simulink model "beaver_agent_env_ground_static_preserved"  (R2022a)
settings: Solver=ode15s  StartTime=0.0  StopTime=30  FixedStep=1/120  MaxStep=0.005  RelTol=1e-6  AbsTol=1e-8
PreLoadFcn:
  | [aircraft, state] = astDehavillandBeaver();
  | thrustX = getCoefficient(aircraft,"CX","Propeller",Component="Propeller");
  | AileronCmd = 0.00202547955338193;
  | ElevatorCmd = -0.0109658218633661;
  | RudderCmd = -0.0374364069557001;
  | Throttle_Left = 0.16863024396043;
  | Throttle_Right = 0.16863024396043;
  | NoseWheelSteerCmdData = timeseries(0,0);
  | GearDownCmd = 1; RunwayMu = 0.65;
  | GroundMass = state.Mass;
  | GroundCrr = 0.015; GroundSideVGain = 0.35;
  | GroundYawGain = 0.15; GroundSteerGain = 0.8; NoseGearArm = 2.4;
  | 
  | Throttle_Left=0; Throttle_Right=0;
  | AileronCmd=0; ElevatorCmd=0; RudderCmd=0;
  | NoseWheelSteerCmdData=timeseries([0;0],[0;60]);
model workspace (MATLAB code in the model file + MAT data in the model file):
  GroundStatic : object (value not decoded)
  inputs0 : object (value not decoded)
  states : object (value not decoded)
  states0 : object (value not decoded)
  other statements: initialize6DOFSkyHogg;
values from neighbouring files (symbols this model uses):
  r = vec(out.r)    [ground_realtime_worker.m]    (also in probe_brake_correction.m; verify_ground_brake_model.m = runCase('turn_right_10',g,10,8))
  state = squeeze(controls.Data)    [finalize_ground_capability_checks.m]    (also in run_ground_capability_checks.m)
symbols that are objects in the model workspace (value not decoded): GroundStatic
undefined symbols (not defined in the file or in its folder): aircraft, Earth, F, Light, MIL, WGS84
libraries: shared6dof x1, aerolibadyn x1, aerolibasang x1, aerolibatmos2 x1, aerolibwind2 x1, aerolibtransform2 x1, sharedtransform x1
(part 2 of 2)

== system beaver_agent_env_ground_static_preserved/GroundContactTireSteering/ThreePointGroundDynamics/LeftMainGear ==
  PositionNED : Inport
  VelocityBody : Inport  Port=2
  AngularRatesBody : Inport  Port=3
  DCMNEDtoBody : Inport  Port=4
  Steering : Inport  Port=5
  GearDown : Inport  Port=6
  RunwayMu : Inport  Port=7
  ParkingBrake : Inport  Port=8
  ContactGeometry : Subsystem
  ContactMoment : Subsystem
  ForceResolution : Subsystem
  NormalReaction : Subsystem
  TireFrictionCircle : Subsystem
  WheelKinematics : Subsystem
  ForceBody : Outport
  MomentBody : Outport  Port=2
  NormalLoad : Outport  Port=3
  Compression : Outport  Port=4
  Contact : Outport  Port=5
  wires:
  ContactMoment/1(AxB) -> MomentBody/1
  ForceResolution/1(BodyForce_1) -> ContactMoment/2(B), ForceBody/1
  PositionNED/1 -> ContactGeometry/1(PositionNED)
  NormalReaction/1(NormalForce_1) -> NormalLoad/1, TireFrictionCircle/6(NormalForce_1), ForceResolution/8(NormalForce), TireFrictionCircle/4(NormalForce)
  AngularRatesBody/1 -> ContactGeometry/5(AngularRatesBody)
  ContactGeometry/5(PositiveCompression_1) -> Compression/1, NormalReaction/3(PositiveCompression)
  NormalReaction/2(ActiveContact_1) -> Contact/1
  ContactGeometry/6(ContactVelocityNED_1) -> WheelKinematics/6(ContactVelocityNED)
  GearDown/1 -> NormalReaction/4(GearDown)
  ContactGeometry/8(ContactGate_1) -> NormalReaction/2(ContactGate)
  ContactGeometry/7(CompressionRate_1) -> NormalReaction/1(CompressionRate)
  ContactGeometry/1(LoadedContactArm_1) -> ContactMoment/1(A)
  Steering/1 -> WheelKinematics/2(Steering)
  ParkingBrake/1 -> TireFrictionCircle/1(ParkingBrake)
  ContactGeometry/2(BodyToNED_1) -> WheelKinematics/3(BodyToNED)
  WheelKinematics/3(WheelLongVelocity_1) -> TireFrictionCircle/2(WheelLongVelocity)
  TireFrictionCircle/2(SideTireForce_1) -> ForceResolution/6(SideTireForce)
  ContactGeometry/3(Zero_1) -> WheelKinematics/4(Zero)
  VelocityBody/1 -> ContactGeometry/4(VelocityBody)
  WheelKinematics/4(WheelSideVelocity_1) -> TireFrictionCircle/3(WheelSideVelocity)
  RunwayMu/1 -> TireFrictionCircle/5(RunwayMu)
  TireFrictionCircle/1(LongTireForce_1) -> ForceResolution/5(LongTireForce)
  WheelKinematics/1(ForwardY_3) -> WheelKinematics/7(ForwardY_2), ForceResolution/7(ForwardY_1), WheelKinematics/1(ForwardY_1), ForceResolution/1(ForwardY)
  WheelKinematics/2(ForwardX_2) -> WheelKinematics/5(ForwardX_1), ForceResolution/2(ForwardX), ForceResolution/4(ForwardX_1)
  DCMNEDtoBody/1 -> ContactGeometry/2(DCMNEDtoBody), ForceResolution/3(DCMNEDtoBody), ContactGeometry/3(DCMNEDtoBody_1)

== system beaver_agent_env_ground_static_preserved/GroundContactTireSteering/ThreePointGroundDynamics/NoseGear ==
  PositionNED : Inport
  VelocityBody : Inport  Port=2
  AngularRatesBody : Inport  Port=3
  DCMNEDtoBody : Inport  Port=4
  Steering : Inport  Port=5
  GearDown : Inport  Port=6
  RunwayMu : Inport  Port=7
  ParkingBrake : Inport  Port=8
  ContactGeometry : Subsystem
  ContactMoment : Subsystem
  ForceResolution : Subsystem
  NormalReaction : Subsystem
  TireFrictionCircle : Subsystem
  WheelKinematics : Subsystem
  ForceBody : Outport
  MomentBody : Outport  Port=2
  NormalLoad : Outport  Port=3
  Compression : Outport  Port=4
  Contact : Outport  Port=5
  wires:
  DCMNEDtoBody/1 -> ContactGeometry/5(DCMNEDtoBody_1), ForceResolution/7(DCMNEDtoBody), ContactGeometry/4(DCMNEDtoBody)
  AngularRatesBody/1 -> ContactGeometry/3(AngularRatesBody)
  ContactMoment/1(AxB) -> MomentBody/1
  ContactGeometry/5(CompressionRate_1) -> NormalReaction/2(CompressionRate)
  PositionNED/1 -> ContactGeometry/1(PositionNED)
  VelocityBody/1 -> ContactGeometry/2(VelocityBody)
  NormalReaction/2(ActiveContact_1) -> Contact/1
  ContactGeometry/6(LoadedContactArm_1) -> ContactMoment/1(A)
  GearDown/1 -> NormalReaction/1(GearDown)
  Steering/1 -> WheelKinematics/2(Steering)
  ContactGeometry/2(ContactVelocityNED_1) -> WheelKinematics/3(ContactVelocityNED)
  ContactGeometry/3(BodyToNED_1) -> WheelKinematics/4(BodyToNED)
  WheelKinematics/1(ForwardY_2) -> ForceResolution/1(ForwardY), WheelKinematics/1(ForwardY_1), ForceResolution/2(ForwardY_1)
  ParkingBrake/1 -> TireFrictionCircle/5(ParkingBrake)
  RunwayMu/1 -> TireFrictionCircle/1(RunwayMu)
  WheelKinematics/3(WheelLongVelocity_1) -> TireFrictionCircle/2(WheelLongVelocity)
  WheelKinematics/4(WheelSideVelocity_1) -> TireFrictionCircle/3(WheelSideVelocity)
  WheelKinematics/2(ForwardX_1) -> ForceResolution/3(ForwardX)
  ContactGeometry/7(ContactGate_1) -> NormalReaction/3(ContactGate)
  ForceResolution/1(BodyForce_1) -> ContactMoment/2(B), ForceBody/1
  ContactGeometry/4(Zero_1) -> WheelKinematics/5(Zero)
  TireFrictionCircle/1(SideTireForce_1) -> ForceResolution/4(SideTireForce)
  TireFrictionCircle/2(LongTireForce_1) -> ForceResolution/5(LongTireForce)
  ContactGeometry/8(PositiveCompression_1) -> NormalReaction/4(PositiveCompression), Compression/1
  NormalReaction/1(NormalForce_1) -> NormalLoad/1, TireFrictionCircle/4(NormalForce), TireFrictionCircle/6(NormalForce_1), ForceResolution/6(NormalForce)

== system beaver_agent_env_ground_static_preserved/GroundContactTireSteering/ThreePointGroundDynamics/RightMainGear ==
  PositionNED : Inport
  VelocityBody : Inport  Port=2
  AngularRatesBody : Inport  Port=3
  DCMNEDtoBody : Inport  Port=4
  Steering : Inport  Port=5
  GearDown : Inport  Port=6
  RunwayMu : Inport  Port=7
  ParkingBrake : Inport  Port=8
  ContactGeometry : Subsystem
  ContactMoment : Subsystem
  ForceResolution : Subsystem
  NormalReaction : Subsystem
  TireFrictionCircle : Subsystem
  WheelKinematics : Subsystem
  ForceBody : Outport
  MomentBody : Outport  Port=2
  NormalLoad : Outport  Port=3
  Compression : Outport  Port=4
  Contact : Outport  Port=5
  wires:
  Steering/1 -> WheelKinematics/2(Steering)
  PositionNED/1 -> ContactGeometry/1(PositionNED)
  GearDown/1 -> NormalReaction/4(GearDown)
  WheelKinematics/1(ForwardY_3) -> WheelKinematics/7(ForwardY_2), ForceResolution/7(ForwardY_1), WheelKinematics/1(ForwardY_1), ForceResolution/1(ForwardY)
  VelocityBody/1 -> ContactGeometry/4(VelocityBody)
  AngularRatesBody/1 -> ContactGeometry/5(AngularRatesBody)
  ContactGeometry/1(LoadedContactArm_1) -> ContactMoment/1(A)
  ContactGeometry/7(CompressionRate_1) -> NormalReaction/1(CompressionRate)
  ContactGeometry/8(ContactGate_1) -> NormalReaction/2(ContactGate)
  NormalReaction/2(ActiveContact_1) -> Contact/1
  TireFrictionCircle/1(LongTireForce_1) -> ForceResolution/5(LongTireForce)
  ContactGeometry/2(BodyToNED_1) -> WheelKinematics/3(BodyToNED)
  ContactGeometry/3(Zero_1) -> WheelKinematics/4(Zero)
  ParkingBrake/1 -> TireFrictionCircle/1(ParkingBrake)
  ContactMoment/1(AxB) -> MomentBody/1
  WheelKinematics/3(WheelLongVelocity_1) -> TireFrictionCircle/2(WheelLongVelocity)
  WheelKinematics/4(WheelSideVelocity_1) -> TireFrictionCircle/3(WheelSideVelocity)
  ContactGeometry/6(ContactVelocityNED_1) -> WheelKinematics/6(ContactVelocityNED)
  TireFrictionCircle/2(SideTireForce_1) -> ForceResolution/6(SideTireForce)
  RunwayMu/1 -> TireFrictionCircle/5(RunwayMu)
  DCMNEDtoBody/1 -> ContactGeometry/2(DCMNEDtoBody), ForceResolution/3(DCMNEDtoBody), ContactGeometry/3(DCMNEDtoBody_1)
  ContactGeometry/5(PositiveCompression_1) -> Compression/1, NormalReaction/3(PositiveCompression)
  WheelKinematics/2(ForwardX_2) -> WheelKinematics/5(ForwardX_1), ForceResolution/2(ForwardX), ForceResolution/4(ForwardX_1)
  ForceResolution/1(BodyForce_1) -> ContactMoment/2(B), ForceBody/1
  NormalReaction/1(NormalForce_1) -> NormalLoad/1, TireFrictionCircle/6(NormalForce_1), ForceResolution/8(NormalForce), TireFrictionCircle/4(NormalForce)

== system beaver_agent_env_ground_static_preserved/Aerodynamic Model/Aerodynamic Coefficients/Body Rate Damping/Subsystem ==
  V : Inport
  Constant1 : Constant  Value=aircraft.ReferenceSpan
  Constant2 : Constant  Value=aircraft.ReferenceLength
  Divide : Subsystem
  Gain1 : Gain  Gain=1/2
  Product : Subsystem
  cV : Outport
  b2V : Outport  Port=2
  wires:
  Product/1(NormalizedRate) -> cV/1
  Constant1/1 -> Gain1/1
  V/1 -> Divide/2(TrueAirspeed), Product/2(TrueAirspeed)
  Divide/1(NormalizedRate) -> b2V/1
  Constant2/1 -> Product/1(Numerator)
  Gain1/1 -> Divide/1(Numerator)

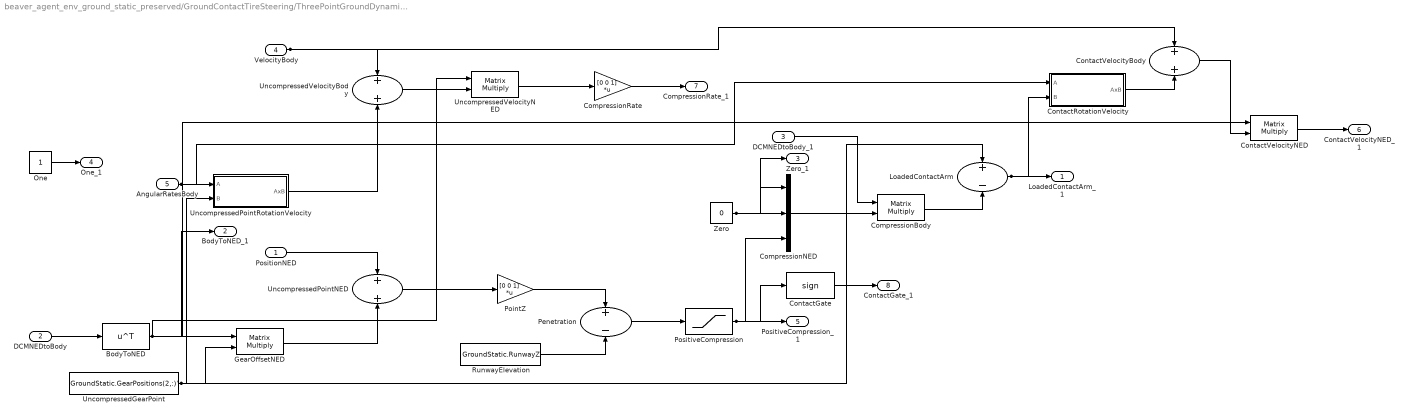
== system beaver_agent_env_ground_static_preserved/GroundContactTireSteering/ThreePointGroundDynamics/LeftMainGear/ContactGeometry ==
  PositionNED : Inport
  DCMNEDtoBody : Inport  Port=2
  DCMNEDtoBody_1 : Inport  Port=3
  VelocityBody : Inport  Port=4
  AngularRatesBody : Inport  Port=5
  BodyToNED : Math  Operator=transpose
  CompressionBody : Product  Inputs=**  Multiplication=Matrix(*)
  CompressionNED : Mux  Inputs=3
  CompressionRate : Gain  Gain=[0 0 1]  Multiplication=Matrix(K*u)
  ContactGate : Signum
  ContactRotationVelocity : Subsystem
  ContactVelocityBody : Sum
  ContactVelocityNED : Product  Inputs=**  Multiplication=Matrix(*)
  GearOffsetNED : Product  Inputs=**  Multiplication=Matrix(*)
  LoadedContactArm : Sum  Inputs=+-
  One : Constant
  Penetration : Sum  Inputs=+-
  PointZ : Gain  Gain=[0 0 1]  Multiplication=Matrix(K*u)
  PositiveCompression : Saturate  UpperLimit=inf  LowerLimit=0
  RunwayElevation : Constant  Value=GroundStatic.RunwayZ
  UncompressedGearPoint : Constant  Value=GroundStatic.GearPositions(2,:)'
  UncompressedPointNED : Sum
  UncompressedPointRotationVelocity : Subsystem
  UncompressedVelocityBody : Sum
  UncompressedVelocityNED : Product  Inputs=**  Multiplication=Matrix(*)
  Zero : Constant  Value=0
  LoadedContactArm_1 : Outport
  BodyToNED_1 : Outport  Port=2
  Zero_1 : Outport  Port=3
  One_1 : Outport  Port=4
  PositiveCompression_1 : Outport  Port=5
  ContactVelocityNED_1 : Outport  Port=6
  CompressionRate_1 : Outport  Port=7
  ContactGate_1 : Outport  Port=8
  wires:
  PositionNED/1 -> UncompressedPointNED/1
  ContactGate/1 -> ContactGate_1/1
  LoadedContactArm/1 -> ContactRotationVelocity/2(B), LoadedContactArm_1/1
  One/1 -> One_1/1
  CompressionRate/1 -> CompressionRate_1/1
  DCMNEDtoBody/1 -> BodyToNED/1
  Penetration/1 -> PositiveCompression/1
  ContactVelocityBody/1 -> ContactVelocityNED/2
  GearOffsetNED/1 -> UncompressedPointNED/2
  DCMNEDtoBody_1/1 -> CompressionBody/1
  UncompressedVelocityNED/1 -> CompressionRate/1
  PositiveCompression/1 -> PositiveCompression_1/1, ContactGate/1, CompressionNED/3
  UncompressedVelocityBody/1 -> UncompressedVelocityNED/2
  ContactRotationVelocity/1(AxB) -> ContactVelocityBody/2
  UncompressedPointRotationVelocity/1(AxB) -> UncompressedVelocityBody/2
  ContactVelocityNED/1 -> ContactVelocityNED_1/1
  UncompressedPointNED/1 -> PointZ/1
  CompressionBody/1 -> LoadedContactArm/2
  CompressionNED/1 -> CompressionBody/2
  PointZ/1 -> Penetration/1
  RunwayElevation/1 -> Penetration/2
  UncompressedGearPoint/1 -> LoadedContactArm/1, GearOffsetNED/2, UncompressedPointRotationVelocity/2(B)
  VelocityBody/1 -> ContactVelocityBody/1, UncompressedVelocityBody/1
  BodyToNED/1 -> ContactVelocityNED/1, GearOffsetNED/1, UncompressedVelocityNED/1, BodyToNED_1/1
  AngularRatesBody/1 -> ContactRotationVelocity/1(A), UncompressedPointRotationVelocity/1(A)
  Zero/1 -> CompressionNED/1, Zero_1/1, CompressionNED/2

== system beaver_agent_env_ground_static_preserved/GroundContactTireSteering/ThreePointGroundDynamics/LeftMainGear/ContactMoment ==
  A : Inport
  B : Inport  Port=2
  C1 : Sum  Inputs=+-
  C2 : Sum  Inputs=+-
  C3 : Sum  Inputs=+-
  DemuxA : Demux  Outputs=3
  DemuxB : Demux  Outputs=3
  N1 : Product  Inputs=**
  N2 : Product  Inputs=**
  N3 : Product  Inputs=**
  P1 : Product  Inputs=**
  P2 : Product  Inputs=**
  P3 : Product  Inputs=**
  Result : Mux  Inputs=3
  AxB : Outport
  wires:
  C1/1 -> Result/1
  Result/1 -> AxB/1
  P3/1 -> C3/1
  B/1 -> DemuxB/1
  C3/1 -> Result/3
  C2/1 -> Result/2
  N3/1 -> C3/2
  N2/1 -> C2/2
  P2/1 -> C2/1
  N1/1 -> C1/2
  P1/1 -> C1/1
  A/1 -> DemuxA/1
  DemuxA/2 -> P1/1, N3/1
  DemuxA/1 -> N2/1, P3/1
  DemuxB/2 -> N1/2, P3/2
  DemuxB/1 -> P2/2, N3/2
  DemuxA/3 -> N1/1, P2/1
  DemuxB/3 -> P1/2, N2/2

== system beaver_agent_env_ground_static_preserved/GroundContactTireSteering/ThreePointGroundDynamics/LeftMainGear/ForceResolution ==
  ForwardY : Inport
  ForwardX : Inport  Port=2
  DCMNEDtoBody : Inport  Port=3
  ForwardX_1 : Inport  Port=4
  LongTireForce : Inport  Port=5
  SideTireForce : Inport  Port=6
  ForwardY_1 : Inport  Port=7
  NormalForce : Inport  Port=8
  BodyForce : Product  Inputs=**  Multiplication=Matrix(*)
  FXLong : Product  Inputs=**
  FXSide : Product  Inputs=**
  FYLong : Product  Inputs=**
  FYSide : Product  Inputs=**
  ForceNED : Mux  Inputs=3
  ForceX : Sum  Inputs=+-
  ForceY : Sum
  ForceZ : Gain  Gain=-1
  BodyForce_1 : Outport
  wires:
  NormalForce/1 -> ForceZ/1
  ForwardY_1/1 -> FYLong/1
  ForwardY/1 -> FXSide/1
  BodyForce/1 -> BodyForce_1/1
  ForwardX/1 -> FXLong/1
  ForwardX_1/1 -> FYSide/1
  FXSide/1 -> ForceX/2
  ForceX/1 -> ForceNED/1
  ForceY/1 -> ForceNED/2
  FXLong/1 -> ForceX/1
  ForceZ/1 -> ForceNED/3
  FYSide/1 -> ForceY/2
  FYLong/1 -> ForceY/1
  LongTireForce/1 -> FYLong/2, FXLong/2
  ForceNED/1 -> BodyForce/2
  DCMNEDtoBody/1 -> BodyForce/1
  SideTireForce/1 -> FXSide/2, FYSide/2

== system beaver_agent_env_ground_static_preserved/GroundContactTireSteering/ThreePointGroundDynamics/LeftMainGear/NormalReaction ==
  CompressionRate : Inport
  ContactGate : Inport  Port=2
  PositiveCompression : Inport  Port=3
  GearDown : Inport  Port=4
  ActiveContact : Product  Inputs=**
  DamperLoad : Gain  Gain=GroundStatic.NormalDamping(2)
  NoTensileNormalForce : Saturate  UpperLimit=inf  LowerLimit=0
  NormalForce : Product  Inputs=***
  SpringDamperLoad : Sum
  SpringLoad : Gain  Gain=GroundStatic.NormalStiffness(2)
  NormalForce_1 : Outport
  ActiveContact_1 : Outport  Port=2
  wires:
  CompressionRate/1 -> DamperLoad/1
  NoTensileNormalForce/1 -> NormalForce/1
  PositiveCompression/1 -> SpringLoad/1
  SpringDamperLoad/1 -> NoTensileNormalForce/1
  NormalForce/1 -> NormalForce_1/1
  ContactGate/1 -> NormalForce/2, ActiveContact/1
  DamperLoad/1 -> SpringDamperLoad/2
  SpringLoad/1 -> SpringDamperLoad/1
  ActiveContact/1 -> ActiveContact_1/1
  GearDown/1 -> ActiveContact/2, NormalForce/3

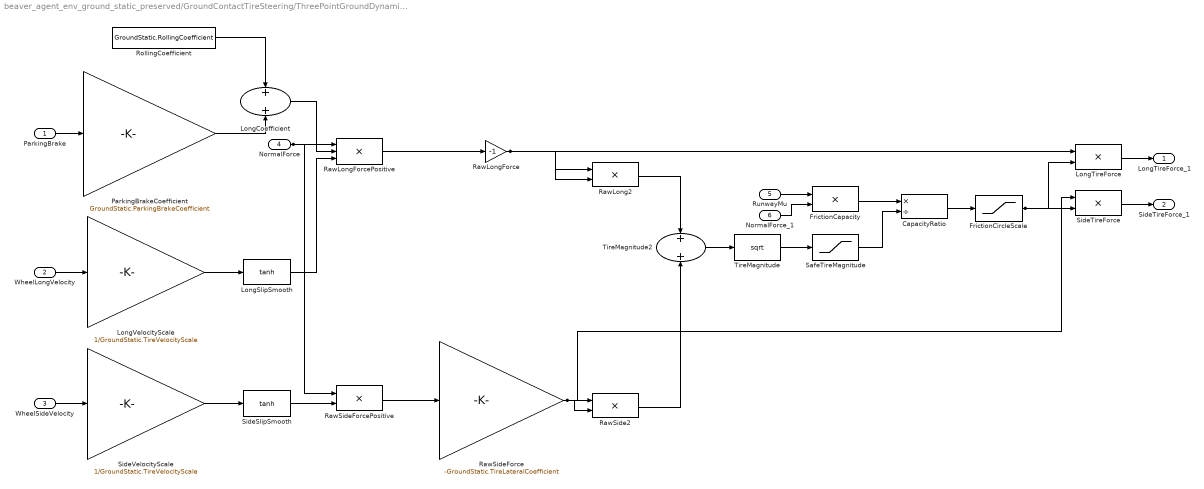
== system beaver_agent_env_ground_static_preserved/GroundContactTireSteering/ThreePointGroundDynamics/LeftMainGear/TireFrictionCircle ==
  ParkingBrake : Inport
  WheelLongVelocity : Inport  Port=2
  WheelSideVelocity : Inport  Port=3
  NormalForce : Inport  Port=4
  RunwayMu : Inport  Port=5
  NormalForce_1 : Inport  Port=6
  CapacityRatio : Product  Inputs=*/
  FrictionCapacity : Product  Inputs=**
  FrictionCircleScale : Saturate  UpperLimit=1  LowerLimit=0
  LongCoefficient : Sum
  LongSlipSmooth : Trigonometry  Operator=tanh
  LongTireForce : Product  Inputs=**
  LongVelocityScale : Gain  Gain=1/GroundStatic.TireVelocityScale
  ParkingBrakeCoefficient : Gain  Gain=GroundStatic.ParkingBrakeCoefficient
  RawLong2 : Product  Inputs=**
  RawLongForce : Gain  Gain=-1
  RawLongForcePositive : Product  Inputs=***
  RawSide2 : Product  Inputs=**
  RawSideForce : Gain  Gain=-GroundStatic.TireLateralCoefficient
  RawSideForcePositive : Product  Inputs=**
  RollingCoefficient : Constant  Value=GroundStatic.RollingCoefficient
  SafeTireMagnitude : Saturate  UpperLimit=inf  LowerLimit=1e-8
  SideSlipSmooth : Trigonometry  Operator=tanh
  SideTireForce : Product  Inputs=**
  SideVelocityScale : Gain  Gain=1/GroundStatic.TireVelocityScale
  TireMagnitude : Sqrt
  TireMagnitude2 : Sum
  LongTireForce_1 : Outport
  SideTireForce_1 : Outport  Port=2
  wires:
  WheelLongVelocity/1 -> LongVelocityScale/1
  LongTireForce/1 -> LongTireForce_1/1
  RunwayMu/1 -> FrictionCapacity/1
  ParkingBrakeCoefficient/1 -> LongCoefficient/2
  RawSide2/1 -> TireMagnitude2/2
  RawSideForcePositive/1 -> RawSideForce/1
  WheelSideVelocity/1 -> SideVelocityScale/1
  LongSlipSmooth/1 -> RawLongForcePositive/3
  RawLongForcePositive/1 -> RawLongForce/1
  SideTireForce/1 -> SideTireForce_1/1
  TireMagnitude2/1 -> TireMagnitude/1
  SideVelocityScale/1 -> SideSlipSmooth/1
  LongCoefficient/1 -> RawLongForcePositive/2
  RollingCoefficient/1 -> LongCoefficient/1
  NormalForce_1/1 -> FrictionCapacity/2
  ParkingBrake/1 -> ParkingBrakeCoefficient/1
  TireMagnitude/1 -> SafeTireMagnitude/1
  SideSlipSmooth/1 -> RawSideForcePositive/2
  RawLong2/1 -> TireMagnitude2/1
  CapacityRatio/1 -> FrictionCircleScale/1
  FrictionCapacity/1 -> CapacityRatio/1
  RawLongForce/1 -> LongTireForce/1, RawLong2/1, RawLong2/2
  LongVelocityScale/1 -> LongSlipSmooth/1
  SafeTireMagnitude/1 -> CapacityRatio/2
  FrictionCircleScale/1 -> SideTireForce/2, LongTireForce/2
  RawSideForce/1 -> SideTireForce/1, RawSide2/2, RawSide2/1
  NormalForce/1 -> RawLongForcePositive/1, RawSideForcePositive/1

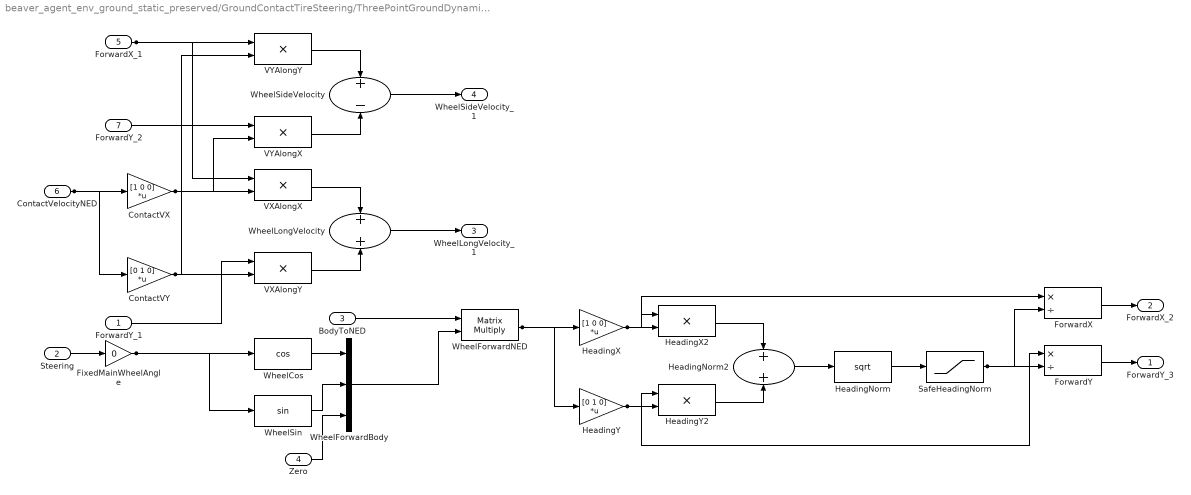
== system beaver_agent_env_ground_static_preserved/GroundContactTireSteering/ThreePointGroundDynamics/LeftMainGear/WheelKinematics ==
  ForwardY_1 : Inport
  Steering : Inport  Port=2
  BodyToNED : Inport  Port=3
  Zero : Inport  Port=4
  ForwardX_1 : Inport  Port=5
  ContactVelocityNED : Inport  Port=6
  ForwardY_2 : Inport  Port=7
  ContactVX : Gain  Gain=[1 0 0]  Multiplication=Matrix(K*u)
  ContactVY : Gain  Gain=[0 1 0]  Multiplication=Matrix(K*u)
  FixedMainWheelAngle : Gain  Gain=0
  ForwardX : Product  Inputs=*/
  ForwardY : Product  Inputs=*/
  HeadingNorm : Sqrt
  HeadingNorm2 : Sum
  HeadingX : Gain  Gain=[1 0 0]  Multiplication=Matrix(K*u)
  HeadingX2 : Product  Inputs=**
  HeadingY : Gain  Gain=[0 1 0]  Multiplication=Matrix(K*u)
  HeadingY2 : Product  Inputs=**
  SafeHeadingNorm : Saturate  UpperLimit=inf  LowerLimit=1e-8
  VXAlongX : Product  Inputs=**
  VXAlongY : Product  Inputs=**
  VYAlongX : Product  Inputs=**
  VYAlongY : Product  Inputs=**
  WheelCos : Trigonometry  Operator=cos
  WheelForwardBody : Mux  Inputs=3
  WheelForwardNED : Product  Inputs=**  Multiplication=Matrix(*)
  WheelLongVelocity : Sum
  WheelSideVelocity : Sum  Inputs=+-
  WheelSin : Trigonometry
  ForwardY_3 : Outport
  ForwardX_2 : Outport  Port=2
  WheelLongVelocity_1 : Outport  Port=3
  WheelSideVelocity_1 : Outport  Port=4
  wires:
  VXAlongX/1 -> WheelLongVelocity/1
  HeadingY/1 -> HeadingY2/2, HeadingY2/1, ForwardY/1
  WheelCos/1 -> WheelForwardBody/1
  Zero/1 -> WheelForwardBody/3
  ForwardY_2/1 -> VYAlongX/1
  HeadingNorm/1 -> SafeHeadingNorm/1
  BodyToNED/1 -> WheelForwardNED/1
  ForwardY/1 -> ForwardY_3/1
  HeadingNorm2/1 -> HeadingNorm/1
  ForwardY_1/1 -> VXAlongY/1
  ForwardX/1 -> ForwardX_2/1
  WheelForwardBody/1 -> WheelForwardNED/2
  HeadingY2/1 -> HeadingNorm2/2
  VYAlongX/1 -> WheelSideVelocity/2
  WheelSin/1 -> WheelForwardBody/2
  WheelLongVelocity/1 -> WheelLongVelocity_1/1
  VXAlongY/1 -> WheelLongVelocity/2
  VYAlongY/1 -> WheelSideVelocity/1
  HeadingX2/1 -> HeadingNorm2/1
  WheelSideVelocity/1 -> WheelSideVelocity_1/1
  Steering/1 -> FixedMainWheelAngle/1
  ContactVY/1 -> VYAlongY/2, VXAlongY/2
  SafeHeadingNorm/1 -> ForwardY/2, ForwardX/2
  WheelForwardNED/1 -> HeadingY/1, HeadingX/1
  ContactVelocityNED/1 -> ContactVY/1, ContactVX/1
  ForwardX_1/1 -> VXAlongX/1, VYAlongY/1
  ContactVX/1 -> VYAlongX/2, VXAlongX/2
  HeadingX/1 -> HeadingX2/2, HeadingX2/1, ForwardX/1
  FixedMainWheelAngle/1 -> WheelSin/1, WheelCos/1

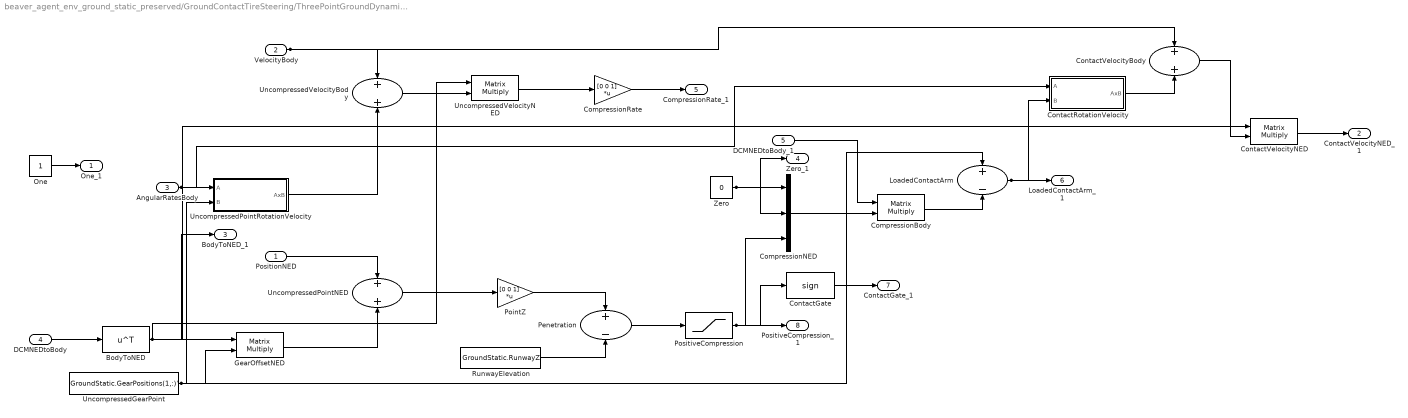
== system beaver_agent_env_ground_static_preserved/GroundContactTireSteering/ThreePointGroundDynamics/NoseGear/ContactGeometry ==
  PositionNED : Inport
  VelocityBody : Inport  Port=2
  AngularRatesBody : Inport  Port=3
  DCMNEDtoBody : Inport  Port=4
  DCMNEDtoBody_1 : Inport  Port=5
  BodyToNED : Math  Operator=transpose
  CompressionBody : Product  Inputs=**  Multiplication=Matrix(*)
  CompressionNED : Mux  Inputs=3
  CompressionRate : Gain  Gain=[0 0 1]  Multiplication=Matrix(K*u)
  ContactGate : Signum
  ContactRotationVelocity : Subsystem
  ContactVelocityBody : Sum
  ContactVelocityNED : Product  Inputs=**  Multiplication=Matrix(*)
  GearOffsetNED : Product  Inputs=**  Multiplication=Matrix(*)
  LoadedContactArm : Sum  Inputs=+-
  One : Constant
  Penetration : Sum  Inputs=+-
  PointZ : Gain  Gain=[0 0 1]  Multiplication=Matrix(K*u)
  PositiveCompression : Saturate  UpperLimit=inf  LowerLimit=0
  RunwayElevation : Constant  Value=GroundStatic.RunwayZ
  UncompressedGearPoint : Constant  Value=GroundStatic.GearPositions(1,:)'
  UncompressedPointNED : Sum
  UncompressedPointRotationVelocity : Subsystem
  UncompressedVelocityBody : Sum
  UncompressedVelocityNED : Product  Inputs=**  Multiplication=Matrix(*)
  Zero : Constant  Value=0
  One_1 : Outport
  ContactVelocityNED_1 : Outport  Port=2
  BodyToNED_1 : Outport  Port=3
  Zero_1 : Outport  Port=4
  CompressionRate_1 : Outport  Port=5
  LoadedContactArm_1 : Outport  Port=6
  ContactGate_1 : Outport  Port=7
  PositiveCompression_1 : Outport  Port=8
  wires:
  CompressionNED/1 -> CompressionBody/2
  PositionNED/1 -> UncompressedPointNED/1
  ContactVelocityNED/1 -> ContactVelocityNED_1/1
  One/1 -> One_1/1
  CompressionRate/1 -> CompressionRate_1/1
  DCMNEDtoBody_1/1 -> CompressionBody/1
  Penetration/1 -> PositiveCompression/1
  CompressionBody/1 -> LoadedContactArm/2
  PointZ/1 -> Penetration/1
  UncompressedVelocityBody/1 -> UncompressedVelocityNED/2
  DCMNEDtoBody/1 -> BodyToNED/1
  GearOffsetNED/1 -> UncompressedPointNED/2
  UncompressedPointNED/1 -> PointZ/1
  ContactGate/1 -> ContactGate_1/1
  UncompressedPointRotationVelocity/1(AxB) -> UncompressedVelocityBody/2
  ContactRotationVelocity/1(AxB) -> ContactVelocityBody/2
  UncompressedVelocityNED/1 -> CompressionRate/1
  ContactVelocityBody/1 -> ContactVelocityNED/2
  RunwayElevation/1 -> Penetration/2
  AngularRatesBody/1 -> ContactRotationVelocity/1(A), UncompressedPointRotationVelocity/1(A)
  VelocityBody/1 -> ContactVelocityBody/1, UncompressedVelocityBody/1
  BodyToNED/1 -> ContactVelocityNED/1, BodyToNED_1/1, UncompressedVelocityNED/1, GearOffsetNED/1
  UncompressedGearPoint/1 -> LoadedContactArm/1, GearOffsetNED/2, UncompressedPointRotationVelocity/2(B)
  LoadedContactArm/1 -> ContactRotationVelocity/2(B), LoadedContactArm_1/1
  PositiveCompression/1 -> CompressionNED/3, PositiveCompression_1/1, ContactGate/1
  Zero/1 -> CompressionNED/2, CompressionNED/1, Zero_1/1

== system beaver_agent_env_ground_static_preserved/GroundContactTireSteering/ThreePointGroundDynamics/NoseGear/ContactMoment ==
  A : Inport
  B : Inport  Port=2
  C1 : Sum  Inputs=+-
  C2 : Sum  Inputs=+-
  C3 : Sum  Inputs=+-
  DemuxA : Demux  Outputs=3
  DemuxB : Demux  Outputs=3
  N1 : Product  Inputs=**
  N2 : Product  Inputs=**
  N3 : Product  Inputs=**
  P1 : Product  Inputs=**
  P2 : Product  Inputs=**
  P3 : Product  Inputs=**
  Result : Mux  Inputs=3
  AxB : Outport
  wires:
  C1/1 -> Result/1
  Result/1 -> AxB/1
  P3/1 -> C3/1
  C3/1 -> Result/3
  C2/1 -> Result/2
  N3/1 -> C3/2
  N2/1 -> C2/2
  P2/1 -> C2/1
  N1/1 -> C1/2
  P1/1 -> C1/1
  B/1 -> DemuxB/1
  A/1 -> DemuxA/1
  DemuxA/1 -> N2/1, P3/1
  DemuxB/1 -> P2/2, N3/2
  DemuxB/3 -> P1/2, N2/2
  DemuxB/2 -> N1/2, P3/2
  DemuxA/2 -> P1/1, N3/1
  DemuxA/3 -> N1/1, P2/1

== system beaver_agent_env_ground_static_preserved/GroundContactTireSteering/ThreePointGroundDynamics/NoseGear/ForceResolution ==
  ForwardY : Inport
  ForwardY_1 : Inport  Port=2
  ForwardX : Inport  Port=3
  SideTireForce : Inport  Port=4
  LongTireForce : Inport  Port=5
  NormalForce : Inport  Port=6
  DCMNEDtoBody : Inport  Port=7
  BodyForce : Product  Inputs=**  Multiplication=Matrix(*)
  FXLong : Product  Inputs=**
  FXSide : Product  Inputs=**
  FYLong : Product  Inputs=**
  FYSide : Product  Inputs=**
  ForceNED : Mux  Inputs=3
  ForceX : Sum  Inputs=+-
  ForceY : Sum
  ForceZ : Gain  Gain=-1
  BodyForce_1 : Outport
  wires:
  ForceNED/1 -> BodyForce/2
  DCMNEDtoBody/1 -> BodyForce/1
  ForwardY/1 -> FXSide/1
  BodyForce/1 -> BodyForce_1/1
  FYLong/1 -> ForceY/1
  NormalForce/1 -> ForceZ/1
  ForceZ/1 -> ForceNED/3
  ForwardY_1/1 -> FYLong/1
  ForceX/1 -> ForceNED/1
  FXSide/1 -> ForceX/2
  ForceY/1 -> ForceNED/2
  FXLong/1 -> ForceX/1
  FYSide/1 -> ForceY/2
  SideTireForce/1 -> FXSide/2, FYSide/2
  ForwardX/1 -> FYSide/1, FXLong/1
  LongTireForce/1 -> FYLong/2, FXLong/2

== system beaver_agent_env_ground_static_preserved/GroundContactTireSteering/ThreePointGroundDynamics/NoseGear/NormalReaction ==
  GearDown : Inport
  CompressionRate : Inport  Port=2
  ContactGate : Inport  Port=3
  PositiveCompression : Inport  Port=4
  ActiveContact : Product  Inputs=**
  DamperLoad : Gain  Gain=GroundStatic.NormalDamping(1)
  NoTensileNormalForce : Saturate  UpperLimit=inf  LowerLimit=0
  NormalForce : Product  Inputs=***
  SpringDamperLoad : Sum
  SpringLoad : Gain  Gain=GroundStatic.NormalStiffness(1)
  NormalForce_1 : Outport
  ActiveContact_1 : Outport  Port=2
  wires:
  CompressionRate/1 -> DamperLoad/1
  NormalForce/1 -> NormalForce_1/1
  NoTensileNormalForce/1 -> NormalForce/1
  ContactGate/1 -> NormalForce/2, ActiveContact/1
  DamperLoad/1 -> SpringDamperLoad/2
  ActiveContact/1 -> ActiveContact_1/1
  PositiveCompression/1 -> SpringLoad/1
  SpringLoad/1 -> SpringDamperLoad/1
  SpringDamperLoad/1 -> NoTensileNormalForce/1
  GearDown/1 -> ActiveContact/2, NormalForce/3

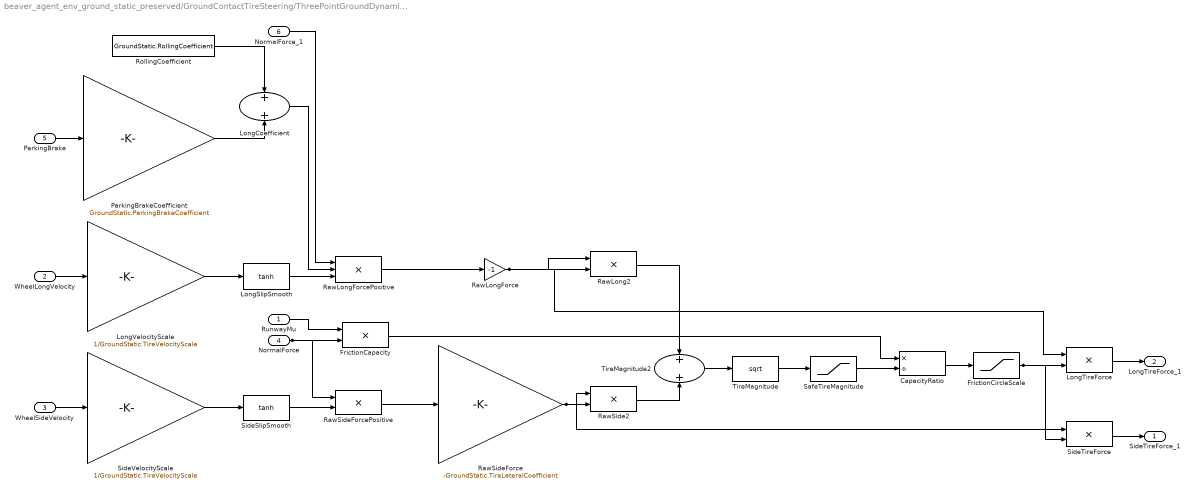
== system beaver_agent_env_ground_static_preserved/GroundContactTireSteering/ThreePointGroundDynamics/NoseGear/TireFrictionCircle ==
  RunwayMu : Inport
  WheelLongVelocity : Inport  Port=2
  WheelSideVelocity : Inport  Port=3
  NormalForce : Inport  Port=4
  ParkingBrake : Inport  Port=5
  NormalForce_1 : Inport  Port=6
  CapacityRatio : Product  Inputs=*/
  FrictionCapacity : Product  Inputs=**
  FrictionCircleScale : Saturate  UpperLimit=1  LowerLimit=0
  LongCoefficient : Sum
  LongSlipSmooth : Trigonometry  Operator=tanh
  LongTireForce : Product  Inputs=**
  LongVelocityScale : Gain  Gain=1/GroundStatic.TireVelocityScale
  ParkingBrakeCoefficient : Gain  Gain=GroundStatic.ParkingBrakeCoefficient
  RawLong2 : Product  Inputs=**
  RawLongForce : Gain  Gain=-1
  RawLongForcePositive : Product  Inputs=***
  RawSide2 : Product  Inputs=**
  RawSideForce : Gain  Gain=-GroundStatic.TireLateralCoefficient
  RawSideForcePositive : Product  Inputs=**
  RollingCoefficient : Constant  Value=GroundStatic.RollingCoefficient
  SafeTireMagnitude : Saturate  UpperLimit=inf  LowerLimit=1e-8
  SideSlipSmooth : Trigonometry  Operator=tanh
  SideTireForce : Product  Inputs=**
  SideVelocityScale : Gain  Gain=1/GroundStatic.TireVelocityScale
  TireMagnitude : Sqrt
  TireMagnitude2 : Sum
  SideTireForce_1 : Outport
  LongTireForce_1 : Outport  Port=2
  wires:
  RawSideForce/1 -> SideTireForce/1, RawSide2/2, RawSide2/1
  ParkingBrake/1 -> ParkingBrakeCoefficient/1
  TireMagnitude/1 -> SafeTireMagnitude/1
  SideTireForce/1 -> SideTireForce_1/1
  WheelLongVelocity/1 -> LongVelocityScale/1
  RunwayMu/1 -> FrictionCapacity/1
  NormalForce_1/1 -> RawLongForcePositive/1
  LongVelocityScale/1 -> LongSlipSmooth/1
  ParkingBrakeCoefficient/1 -> LongCoefficient/2
  RollingCoefficient/1 -> LongCoefficient/1
  RawSide2/1 -> TireMagnitude2/2
  FrictionCapacity/1 -> CapacityRatio/1
  LongCoefficient/1 -> RawLongForcePositive/2
  LongTireForce/1 -> LongTireForce_1/1
  SafeTireMagnitude/1 -> CapacityRatio/2
  TireMagnitude2/1 -> TireMagnitude/1
  RawSideForcePositive/1 -> RawSideForce/1
  RawLongForcePositive/1 -> RawLongForce/1
  CapacityRatio/1 -> FrictionCircleScale/1
  SideSlipSmooth/1 -> RawSideForcePositive/2
  LongSlipSmooth/1 -> RawLongForcePositive/3
  WheelSideVelocity/1 -> SideVelocityScale/1
  SideVelocityScale/1 -> SideSlipSmooth/1
  RawLong2/1 -> TireMagnitude2/1
  FrictionCircleScale/1 -> SideTireForce/2, LongTireForce/2
  RawLongForce/1 -> LongTireForce/1, RawLong2/1, RawLong2/2
  NormalForce/1 -> RawSideForcePositive/1, FrictionCapacity/2

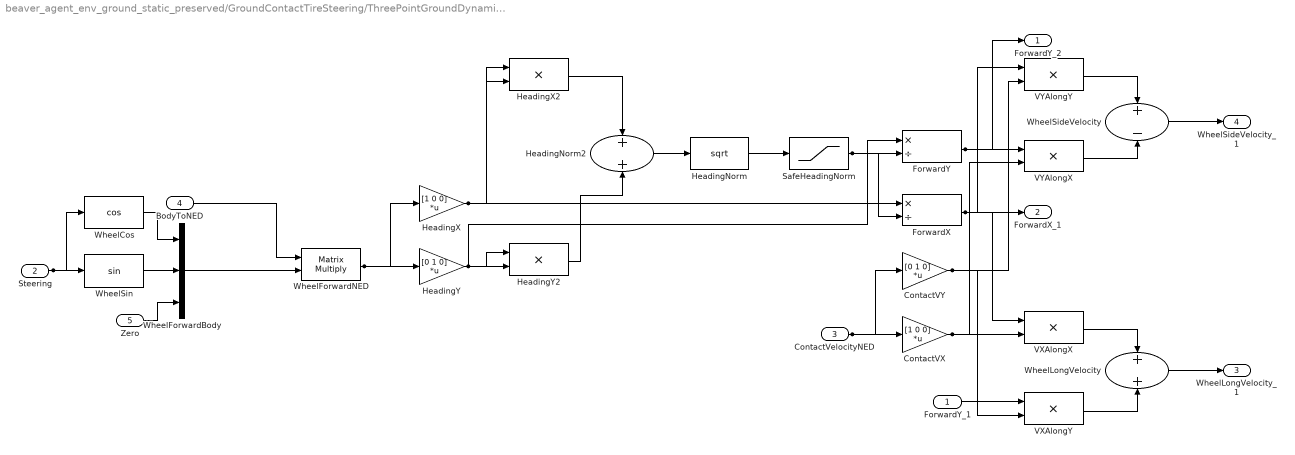
== system beaver_agent_env_ground_static_preserved/GroundContactTireSteering/ThreePointGroundDynamics/NoseGear/WheelKinematics ==
  ForwardY_1 : Inport
  Steering : Inport  Port=2
  ContactVelocityNED : Inport  Port=3
  BodyToNED : Inport  Port=4
  Zero : Inport  Port=5
  ContactVX : Gain  Gain=[1 0 0]  Multiplication=Matrix(K*u)
  ContactVY : Gain  Gain=[0 1 0]  Multiplication=Matrix(K*u)
  ForwardX : Product  Inputs=*/
  ForwardY : Product  Inputs=*/
  HeadingNorm : Sqrt
  HeadingNorm2 : Sum
  HeadingX : Gain  Gain=[1 0 0]  Multiplication=Matrix(K*u)
  HeadingX2 : Product  Inputs=**
  HeadingY : Gain  Gain=[0 1 0]  Multiplication=Matrix(K*u)
  HeadingY2 : Product  Inputs=**
  SafeHeadingNorm : Saturate  UpperLimit=inf  LowerLimit=1e-8
  VXAlongX : Product  Inputs=**
  VXAlongY : Product  Inputs=**
  VYAlongX : Product  Inputs=**
  VYAlongY : Product  Inputs=**
  WheelCos : Trigonometry  Operator=cos
  WheelForwardBody : Mux  Inputs=3
  WheelForwardNED : Product  Inputs=**  Multiplication=Matrix(*)
  WheelLongVelocity : Sum
  WheelSideVelocity : Sum  Inputs=+-
  WheelSin : Trigonometry
  ForwardY_2 : Outport
  ForwardX_1 : Outport  Port=2
  WheelLongVelocity_1 : Outport  Port=3
  WheelSideVelocity_1 : Outport  Port=4
  wires:
  Zero/1 -> WheelForwardBody/3
  HeadingNorm2/1 -> HeadingNorm/1
  VXAlongY/1 -> WheelLongVelocity/2
  VXAlongX/1 -> WheelLongVelocity/1
  WheelForwardBody/1 -> WheelForwardNED/2
  WheelCos/1 -> WheelForwardBody/1
  BodyToNED/1 -> WheelForwardNED/1
  WheelSin/1 -> WheelForwardBody/2
  WheelLongVelocity/1 -> WheelLongVelocity_1/1
  HeadingY2/1 -> HeadingNorm2/2
  HeadingNorm/1 -> SafeHeadingNorm/1
  WheelSideVelocity/1 -> WheelSideVelocity_1/1
  HeadingX2/1 -> HeadingNorm2/1
  VYAlongY/1 -> WheelSideVelocity/1
  ContactVX/1 -> VYAlongX/2, VXAlongX/2
  ForwardY_1/1 -> VXAlongY/1
  VYAlongX/1 -> WheelSideVelocity/2
  ContactVelocityNED/1 -> ContactVX/1, ContactVY/1
  HeadingX/1 -> ForwardX/1, HeadingX2/1, HeadingX2/2
  Steering/1 -> WheelSin/1, WheelCos/1
  HeadingY/1 -> ForwardY/1, HeadingY2/1, HeadingY2/2
  ContactVY/1 -> VYAlongY/2, VXAlongY/2
  SafeHeadingNorm/1 -> ForwardY/2, ForwardX/2
  ForwardY/1 -> VYAlongX/1, ForwardY_2/1
  ForwardX/1 -> VXAlongX/1, ForwardX_1/1, VYAlongY/1
  WheelForwardNED/1 -> HeadingY/1, HeadingX/1

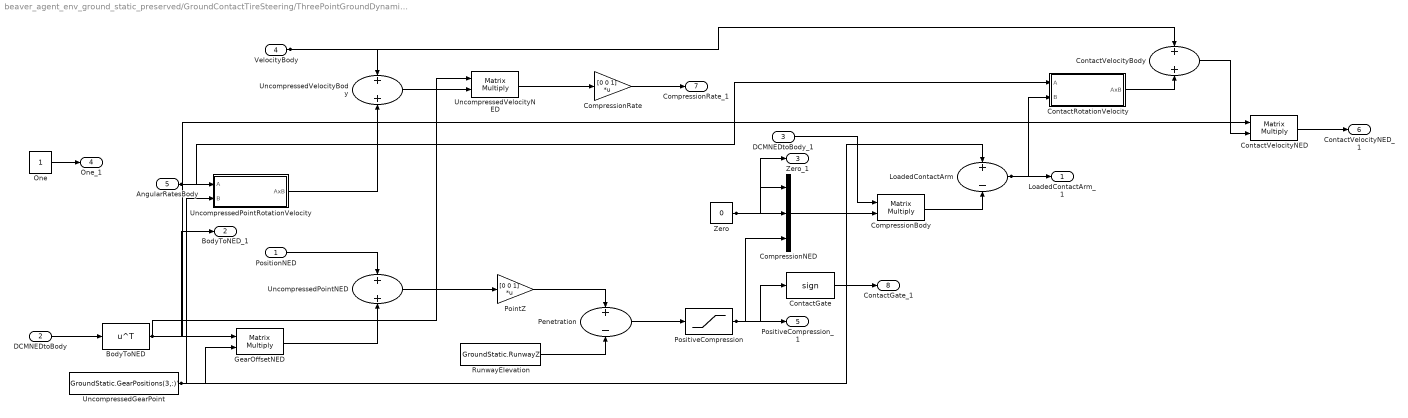
== system beaver_agent_env_ground_static_preserved/GroundContactTireSteering/ThreePointGroundDynamics/RightMainGear/ContactGeometry ==
  PositionNED : Inport
  DCMNEDtoBody : Inport  Port=2
  DCMNEDtoBody_1 : Inport  Port=3
  VelocityBody : Inport  Port=4
  AngularRatesBody : Inport  Port=5
  BodyToNED : Math  Operator=transpose
  CompressionBody : Product  Inputs=**  Multiplication=Matrix(*)
  CompressionNED : Mux  Inputs=3
  CompressionRate : Gain  Gain=[0 0 1]  Multiplication=Matrix(K*u)
  ContactGate : Signum
  ContactRotationVelocity : Subsystem
  ContactVelocityBody : Sum
  ContactVelocityNED : Product  Inputs=**  Multiplication=Matrix(*)
  GearOffsetNED : Product  Inputs=**  Multiplication=Matrix(*)
  LoadedContactArm : Sum  Inputs=+-
  One : Constant
  Penetration : Sum  Inputs=+-
  PointZ : Gain  Gain=[0 0 1]  Multiplication=Matrix(K*u)
  PositiveCompression : Saturate  UpperLimit=inf  LowerLimit=0
  RunwayElevation : Constant  Value=GroundStatic.RunwayZ
  UncompressedGearPoint : Constant  Value=GroundStatic.GearPositions(3,:)'
  UncompressedPointNED : Sum
  UncompressedPointRotationVelocity : Subsystem
  UncompressedVelocityBody : Sum
  UncompressedVelocityNED : Product  Inputs=**  Multiplication=Matrix(*)
  Zero : Constant  Value=0
  LoadedContactArm_1 : Outport
  BodyToNED_1 : Outport  Port=2
  Zero_1 : Outport  Port=3
  One_1 : Outport  Port=4
  PositiveCompression_1 : Outport  Port=5
  ContactVelocityNED_1 : Outport  Port=6
  CompressionRate_1 : Outport  Port=7
  ContactGate_1 : Outport  Port=8
  wires:
  RunwayElevation/1 -> Penetration/2
  PositionNED/1 -> UncompressedPointNED/1
  LoadedContactArm/1 -> ContactRotationVelocity/2(B), LoadedContactArm_1/1
  CompressionRate/1 -> CompressionRate_1/1
  DCMNEDtoBody_1/1 -> CompressionBody/1
  Penetration/1 -> PositiveCompression/1
  DCMNEDtoBody/1 -> BodyToNED/1
  ContactVelocityBody/1 -> ContactVelocityNED/2
  One/1 -> One_1/1
  ContactRotationVelocity/1(AxB) -> ContactVelocityBody/2
  ContactGate/1 -> ContactGate_1/1
  UncompressedPointNED/1 -> PointZ/1
  UncompressedVelocityBody/1 -> UncompressedVelocityNED/2
  UncompressedVelocityNED/1 -> CompressionRate/1
  CompressionBody/1 -> LoadedContactArm/2
  PointZ/1 -> Penetration/1
  GearOffsetNED/1 -> UncompressedPointNED/2
  CompressionNED/1 -> CompressionBody/2
  UncompressedPointRotationVelocity/1(AxB) -> UncompressedVelocityBody/2
  ContactVelocityNED/1 -> ContactVelocityNED_1/1
  AngularRatesBody/1 -> ContactRotationVelocity/1(A), UncompressedPointRotationVelocity/1(A)
  PositiveCompression/1 -> PositiveCompression_1/1, ContactGate/1, CompressionNED/3
  VelocityBody/1 -> ContactVelocityBody/1, UncompressedVelocityBody/1
  UncompressedGearPoint/1 -> LoadedContactArm/1, GearOffsetNED/2, UncompressedPointRotationVelocity/2(B)
  Zero/1 -> CompressionNED/1, Zero_1/1, CompressionNED/2
  BodyToNED/1 -> ContactVelocityNED/1, GearOffsetNED/1, UncompressedVelocityNED/1, BodyToNED_1/1

== system beaver_agent_env_ground_static_preserved/GroundContactTireSteering/ThreePointGroundDynamics/RightMainGear/ContactMoment ==
  A : Inport
  B : Inport  Port=2
  C1 : Sum  Inputs=+-
  C2 : Sum  Inputs=+-
  C3 : Sum  Inputs=+-
  DemuxA : Demux  Outputs=3
  DemuxB : Demux  Outputs=3
  N1 : Product  Inputs=**
  N2 : Product  Inputs=**
  N3 : Product  Inputs=**
  P1 : Product  Inputs=**
  P2 : Product  Inputs=**
  P3 : Product  Inputs=**
  Result : Mux  Inputs=3
  AxB : Outport
  wires:
  C1/1 -> Result/1
  Result/1 -> AxB/1
  P3/1 -> C3/1
  C3/1 -> Result/3
  C2/1 -> Result/2
  N3/1 -> C3/2
  N2/1 -> C2/2
  P2/1 -> C2/1
  N1/1 -> C1/2
  P1/1 -> C1/1
  B/1 -> DemuxB/1
  A/1 -> DemuxA/1
  DemuxA/1 -> N2/1, P3/1
  DemuxB/1 -> P2/2, N3/2
  DemuxB/3 -> P1/2, N2/2
  DemuxB/2 -> N1/2, P3/2
  DemuxA/2 -> P1/1, N3/1
  DemuxA/3 -> N1/1, P2/1

== system beaver_agent_env_ground_static_preserved/GroundContactTireSteering/ThreePointGroundDynamics/RightMainGear/ForceResolution ==
  ForwardY : Inport
  ForwardX : Inport  Port=2
  DCMNEDtoBody : Inport  Port=3
  ForwardX_1 : Inport  Port=4
  LongTireForce : Inport  Port=5
  SideTireForce : Inport  Port=6
  ForwardY_1 : Inport  Port=7
  NormalForce : Inport  Port=8
  BodyForce : Product  Inputs=**  Multiplication=Matrix(*)
  FXLong : Product  Inputs=**
  FXSide : Product  Inputs=**
  FYLong : Product  Inputs=**
  FYSide : Product  Inputs=**
  ForceNED : Mux  Inputs=3
  ForceX : Sum  Inputs=+-
  ForceY : Sum
  ForceZ : Gain  Gain=-1
  BodyForce_1 : Outport
  wires:
  ForwardY/1 -> FXSide/1
  DCMNEDtoBody/1 -> BodyForce/1
  BodyForce/1 -> BodyForce_1/1
  ForwardX/1 -> FXLong/1
  FYSide/1 -> ForceY/2
  NormalForce/1 -> ForceZ/1
  ForwardY_1/1 -> FYLong/1
  ForwardX_1/1 -> FYSide/1
  ForceZ/1 -> ForceNED/3
  ForceNED/1 -> BodyForce/2
  FXLong/1 -> ForceX/1
  ForceY/1 -> ForceNED/2
  FXSide/1 -> ForceX/2
  ForceX/1 -> ForceNED/1
  FYLong/1 -> ForceY/1
  LongTireForce/1 -> FYLong/2, FXLong/2
  SideTireForce/1 -> FXSide/2, FYSide/2

== system beaver_agent_env_ground_static_preserved/GroundContactTireSteering/ThreePointGroundDynamics/RightMainGear/NormalReaction ==
  CompressionRate : Inport
  ContactGate : Inport  Port=2
  PositiveCompression : Inport  Port=3
  GearDown : Inport  Port=4
  ActiveContact : Product  Inputs=**
  DamperLoad : Gain  Gain=GroundStatic.NormalDamping(3)
  NoTensileNormalForce : Saturate  UpperLimit=inf  LowerLimit=0
  NormalForce : Product  Inputs=***
  SpringDamperLoad : Sum
  SpringLoad : Gain  Gain=GroundStatic.NormalStiffness(3)
  NormalForce_1 : Outport
  ActiveContact_1 : Outport  Port=2
  wires:
  ActiveContact/1 -> ActiveContact_1/1
  DamperLoad/1 -> SpringDamperLoad/2
  PositiveCompression/1 -> SpringLoad/1
  SpringDamperLoad/1 -> NoTensileNormalForce/1
  NormalForce/1 -> NormalForce_1/1
  CompressionRate/1 -> DamperLoad/1
  SpringLoad/1 -> SpringDamperLoad/1
  NoTensileNormalForce/1 -> NormalForce/1
  ContactGate/1 -> ActiveContact/1, NormalForce/2
  GearDown/1 -> ActiveContact/2, NormalForce/3

== system beaver_agent_env_ground_static_preserved/GroundContactTireSteering/ThreePointGroundDynamics/RightMainGear/TireFrictionCircle ==
  ParkingBrake : Inport
  WheelLongVelocity : Inport  Port=2
  WheelSideVelocity : Inport  Port=3
  NormalForce : Inport  Port=4
  RunwayMu : Inport  Port=5
  NormalForce_1 : Inport  Port=6
  CapacityRatio : Product  Inputs=*/
  FrictionCapacity : Product  Inputs=**
  FrictionCircleScale : Saturate  UpperLimit=1  LowerLimit=0
  LongCoefficient : Sum
  LongSlipSmooth : Trigonometry  Operator=tanh
  LongTireForce : Product  Inputs=**
  LongVelocityScale : Gain  Gain=1/GroundStatic.TireVelocityScale
  ParkingBrakeCoefficient : Gain  Gain=GroundStatic.ParkingBrakeCoefficient
  RawLong2 : Product  Inputs=**
  RawLongForce : Gain  Gain=-1
  RawLongForcePositive : Product  Inputs=***
  RawSide2 : Product  Inputs=**
  RawSideForce : Gain  Gain=-GroundStatic.TireLateralCoefficient
  RawSideForcePositive : Product  Inputs=**
  RollingCoefficient : Constant  Value=GroundStatic.RollingCoefficient
  SafeTireMagnitude : Saturate  UpperLimit=inf  LowerLimit=1e-8
  SideSlipSmooth : Trigonometry  Operator=tanh
  SideTireForce : Product  Inputs=**
  SideVelocityScale : Gain  Gain=1/GroundStatic.TireVelocityScale
  TireMagnitude : Sqrt
  TireMagnitude2 : Sum
  LongTireForce_1 : Outport
  SideTireForce_1 : Outport  Port=2
  wires:
  SideTireForce/1 -> SideTireForce_1/1
  RawLongForce/1 -> LongTireForce/1, RawLong2/1, RawLong2/2
  NormalForce_1/1 -> FrictionCapacity/2
  SafeTireMagnitude/1 -> CapacityRatio/2
  FrictionCircleScale/1 -> SideTireForce/2, LongTireForce/2
  RunwayMu/1 -> FrictionCapacity/1
  WheelLongVelocity/1 -> LongVelocityScale/1
  LongTireForce/1 -> LongTireForce_1/1
  LongVelocityScale/1 -> LongSlipSmooth/1
  FrictionCapacity/1 -> CapacityRatio/1
  TireMagnitude/1 -> SafeTireMagnitude/1
  ParkingBrakeCoefficient/1 -> LongCoefficient/2
  RawLongForcePositive/1 -> RawLongForce/1
  LongSlipSmooth/1 -> RawLongForcePositive/3
  WheelSideVelocity/1 -> SideVelocityScale/1
  LongCoefficient/1 -> RawLongForcePositive/2
  RawLong2/1 -> TireMagnitude2/1
  RawSideForcePositive/1 -> RawSideForce/1
  CapacityRatio/1 -> FrictionCircleScale/1
  SideSlipSmooth/1 -> RawSideForcePositive/2
  TireMagnitude2/1 -> TireMagnitude/1
  RawSide2/1 -> TireMagnitude2/2
  NormalForce/1 -> RawLongForcePositive/1, RawSideForcePositive/1
  RollingCoefficient/1 -> LongCoefficient/1
  SideVelocityScale/1 -> SideSlipSmooth/1
  ParkingBrake/1 -> ParkingBrakeCoefficient/1
  RawSideForce/1 -> SideTireForce/1, RawSide2/2, RawSide2/1

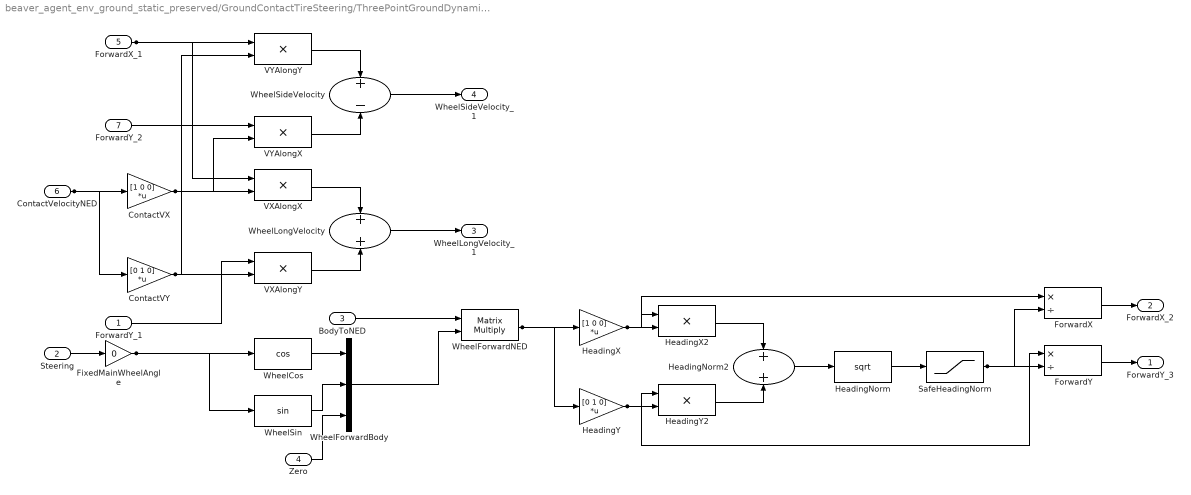
== system beaver_agent_env_ground_static_preserved/GroundContactTireSteering/ThreePointGroundDynamics/RightMainGear/WheelKinematics ==
  ForwardY_1 : Inport
  Steering : Inport  Port=2
  BodyToNED : Inport  Port=3
  Zero : Inport  Port=4
  ForwardX_1 : Inport  Port=5
  ContactVelocityNED : Inport  Port=6
  ForwardY_2 : Inport  Port=7
  ContactVX : Gain  Gain=[1 0 0]  Multiplication=Matrix(K*u)
  ContactVY : Gain  Gain=[0 1 0]  Multiplication=Matrix(K*u)
  FixedMainWheelAngle : Gain  Gain=0
  ForwardX : Product  Inputs=*/
  ForwardY : Product  Inputs=*/
  HeadingNorm : Sqrt
  HeadingNorm2 : Sum
  HeadingX : Gain  Gain=[1 0 0]  Multiplication=Matrix(K*u)
  HeadingX2 : Product  Inputs=**
  HeadingY : Gain  Gain=[0 1 0]  Multiplication=Matrix(K*u)
  HeadingY2 : Product  Inputs=**
  SafeHeadingNorm : Saturate  UpperLimit=inf  LowerLimit=1e-8
  VXAlongX : Product  Inputs=**
  VXAlongY : Product  Inputs=**
  VYAlongX : Product  Inputs=**
  VYAlongY : Product  Inputs=**
  WheelCos : Trigonometry  Operator=cos
  WheelForwardBody : Mux  Inputs=3
  WheelForwardNED : Product  Inputs=**  Multiplication=Matrix(*)
  WheelLongVelocity : Sum
  WheelSideVelocity : Sum  Inputs=+-
  WheelSin : Trigonometry
  ForwardY_3 : Outport
  ForwardX_2 : Outport  Port=2
  WheelLongVelocity_1 : Outport  Port=3
  WheelSideVelocity_1 : Outport  Port=4
  wires:
  BodyToNED/1 -> WheelForwardNED/1
  WheelLongVelocity/1 -> WheelLongVelocity_1/1
  SafeHeadingNorm/1 -> ForwardY/2, ForwardX/2
  ContactVY/1 -> VYAlongY/2, VXAlongY/2
  Zero/1 -> WheelForwardBody/3
  ContactVelocityNED/1 -> ContactVY/1, ContactVX/1
  WheelSideVelocity/1 -> WheelSideVelocity_1/1
  WheelSin/1 -> WheelForwardBody/2
  ForwardY/1 -> ForwardY_3/1
  VXAlongY/1 -> WheelLongVelocity/2
  ForwardX_1/1 -> VYAlongY/1, VXAlongX/1
  HeadingX2/1 -> HeadingNorm2/1
  WheelForwardBody/1 -> WheelForwardNED/2
  VYAlongY/1 -> WheelSideVelocity/1
  ForwardY_1/1 -> VXAlongY/1
  VXAlongX/1 -> WheelLongVelocity/1
  HeadingNorm2/1 -> HeadingNorm/1
  ForwardY_2/1 -> VYAlongX/1
  WheelCos/1 -> WheelForwardBody/1
  Steering/1 -> FixedMainWheelAngle/1
  HeadingY2/1 -> HeadingNorm2/2
  VYAlongX/1 -> WheelSideVelocity/2
  HeadingNorm/1 -> SafeHeadingNorm/1
  ForwardX/1 -> ForwardX_2/1
  FixedMainWheelAngle/1 -> WheelSin/1, WheelCos/1
  WheelForwardNED/1 -> HeadingY/1, HeadingX/1
  HeadingX/1 -> HeadingX2/2, HeadingX2/1, ForwardX/1
  HeadingY/1 -> HeadingY2/2, HeadingY2/1, ForwardY/1
  ContactVX/1 -> VYAlongX/2, VXAlongX/2

== system beaver_agent_env_ground_static_preserved/Aerodynamic Model/Aerodynamic Coefficients/Body Rate Damping/Subsystem/Divide ==
  Numerator : Inport
  TrueAirspeed : Inport  Port=2
  NonzeroAirspeed : Saturate  UpperLimit=inf  LowerLimit=GroundStatic.AirSpeedFloor
  OriginalDivision : Product  Inputs=*/
  NormalizedRate : Outport
  wires:
  TrueAirspeed/1 -> NonzeroAirspeed/1
  OriginalDivision/1 -> NormalizedRate/1
  NonzeroAirspeed/1 -> OriginalDivision/2
  Numerator/1 -> OriginalDivision/1

== system beaver_agent_env_ground_static_preserved/Aerodynamic Model/Aerodynamic Coefficients/Body Rate Damping/Subsystem/Product ==
  Numerator : Inport
  TrueAirspeed : Inport  Port=2
  NonzeroAirspeed : Saturate  UpperLimit=inf  LowerLimit=GroundStatic.AirSpeedFloor
  OriginalDivision : Product  Inputs=*/
  NormalizedRate : Outport
  wires:
  TrueAirspeed/1 -> NonzeroAirspeed/1
  OriginalDivision/1 -> NormalizedRate/1
  Numerator/1 -> OriginalDivision/1
  NonzeroAirspeed/1 -> OriginalDivision/2

== system beaver_agent_env_ground_static_preserved/GroundContactTireSteering/ThreePointGroundDynamics/LeftMainGear/ContactGeometry/ContactRotationVelocity ==
  A : Inport
  B : Inport  Port=2
  C1 : Sum  Inputs=+-
  C2 : Sum  Inputs=+-
  C3 : Sum  Inputs=+-
  DemuxA : Demux  Outputs=3
  DemuxB : Demux  Outputs=3
  N1 : Product  Inputs=**
  N2 : Product  Inputs=**
  N3 : Product  Inputs=**
  P1 : Product  Inputs=**
  P2 : Product  Inputs=**
  P3 : Product  Inputs=**
  Result : Mux  Inputs=3
  AxB : Outport
  wires:
  C1/1 -> Result/1
  Result/1 -> AxB/1
  P3/1 -> C3/1
  C3/1 -> Result/3
  C2/1 -> Result/2
  N3/1 -> C3/2
  N2/1 -> C2/2
  P2/1 -> C2/1
  N1/1 -> C1/2
  P1/1 -> C1/1
  B/1 -> DemuxB/1
  A/1 -> DemuxA/1
  DemuxA/1 -> N2/1, P3/1
  DemuxB/1 -> P2/2, N3/2
  DemuxB/3 -> P1/2, N2/2
  DemuxB/2 -> N1/2, P3/2
  DemuxA/2 -> P1/1, N3/1
  DemuxA/3 -> N1/1, P2/1

== system beaver_agent_env_ground_static_preserved/GroundContactTireSteering/ThreePointGroundDynamics/LeftMainGear/ContactGeometry/UncompressedPointRotationVelocity ==
  A : Inport
  B : Inport  Port=2
  C1 : Sum  Inputs=+-
  C2 : Sum  Inputs=+-
  C3 : Sum  Inputs=+-
  DemuxA : Demux  Outputs=3
  DemuxB : Demux  Outputs=3
  N1 : Product  Inputs=**
  N2 : Product  Inputs=**
  N3 : Product  Inputs=**
  P1 : Product  Inputs=**
  P2 : Product  Inputs=**
  P3 : Product  Inputs=**
  Result : Mux  Inputs=3
  AxB : Outport
  wires:
  P2/1 -> C2/1
  C1/1 -> Result/1
  Result/1 -> AxB/1
  DemuxA/2 -> P1/1, N3/1
  P3/1 -> C3/1
  N1/1 -> C1/2
  C3/1 -> Result/3
  DemuxA/1 -> N2/1, P3/1
  C2/1 -> Result/2
  N3/1 -> C3/2
  N2/1 -> C2/2
  P1/1 -> C1/1
  B/1 -> DemuxB/1
  A/1 -> DemuxA/1
  DemuxB/1 -> P2/2, N3/2
  DemuxB/3 -> P1/2, N2/2
  DemuxB/2 -> N1/2, P3/2
  DemuxA/3 -> N1/1, P2/1

== system beaver_agent_env_ground_static_preserved/GroundContactTireSteering/ThreePointGroundDynamics/NoseGear/ContactGeometry/ContactRotationVelocity ==
  A : Inport
  B : Inport  Port=2
  C1 : Sum  Inputs=+-
  C2 : Sum  Inputs=+-
  C3 : Sum  Inputs=+-
  DemuxA : Demux  Outputs=3
  DemuxB : Demux  Outputs=3
  N1 : Product  Inputs=**
  N2 : Product  Inputs=**
  N3 : Product  Inputs=**
  P1 : Product  Inputs=**
  P2 : Product  Inputs=**
  P3 : Product  Inputs=**
  Result : Mux  Inputs=3
  AxB : Outport
  wires:
  C1/1 -> Result/1
  Result/1 -> AxB/1
  P3/1 -> C3/1
  B/1 -> DemuxB/1
  C3/1 -> Result/3
  C2/1 -> Result/2
  N3/1 -> C3/2
  N2/1 -> C2/2
  P2/1 -> C2/1
  N1/1 -> C1/2
  P1/1 -> C1/1
  A/1 -> DemuxA/1
  DemuxA/2 -> P1/1, N3/1
  DemuxA/1 -> N2/1, P3/1
  DemuxB/2 -> N1/2, P3/2
  DemuxB/1 -> P2/2, N3/2
  DemuxA/3 -> N1/1, P2/1
  DemuxB/3 -> P1/2, N2/2

== system beaver_agent_env_ground_static_preserved/GroundContactTireSteering/ThreePointGroundDynamics/NoseGear/ContactGeometry/UncompressedPointRotationVelocity ==
  A : Inport
  B : Inport  Port=2
  C1 : Sum  Inputs=+-
  C2 : Sum  Inputs=+-
  C3 : Sum  Inputs=+-
  DemuxA : Demux  Outputs=3
  DemuxB : Demux  Outputs=3
  N1 : Product  Inputs=**
  N2 : Product  Inputs=**
  N3 : Product  Inputs=**
  P1 : Product  Inputs=**
  P2 : Product  Inputs=**
  P3 : Product  Inputs=**
  Result : Mux  Inputs=3
  AxB : Outport
  wires:
  C1/1 -> Result/1
  Result/1 -> AxB/1
  P3/1 -> C3/1
  C3/1 -> Result/3
  C2/1 -> Result/2
  N3/1 -> C3/2
  N2/1 -> C2/2
  P2/1 -> C2/1
  N1/1 -> C1/2
  P1/1 -> C1/1
  B/1 -> DemuxB/1
  A/1 -> DemuxA/1
  DemuxA/1 -> N2/1, P3/1
  DemuxB/1 -> P2/2, N3/2
  DemuxB/3 -> P1/2, N2/2
  DemuxB/2 -> N1/2, P3/2
  DemuxA/2 -> P1/1, N3/1
  DemuxA/3 -> N1/1, P2/1

== system beaver_agent_env_ground_static_preserved/GroundContactTireSteering/ThreePointGroundDynamics/RightMainGear/ContactGeometry/ContactRotationVelocity ==
  A : Inport
  B : Inport  Port=2
  C1 : Sum  Inputs=+-
  C2 : Sum  Inputs=+-
  C3 : Sum  Inputs=+-
  DemuxA : Demux  Outputs=3
  DemuxB : Demux  Outputs=3
  N1 : Product  Inputs=**
  N2 : Product  Inputs=**
  N3 : Product  Inputs=**
  P1 : Product  Inputs=**
  P2 : Product  Inputs=**
  P3 : Product  Inputs=**
  Result : Mux  Inputs=3
  AxB : Outport
  wires:
  C1/1 -> Result/1
  Result/1 -> AxB/1
  P3/1 -> C3/1
  C3/1 -> Result/3
  C2/1 -> Result/2
  N3/1 -> C3/2
  N2/1 -> C2/2
  P2/1 -> C2/1
  N1/1 -> C1/2
  P1/1 -> C1/1
  B/1 -> DemuxB/1
  A/1 -> DemuxA/1
  DemuxA/2 -> P1/1, N3/1
  DemuxA/1 -> N2/1, P3/1
  DemuxB/2 -> N1/2, P3/2
  DemuxB/1 -> P2/2, N3/2
  DemuxA/3 -> N1/1, P2/1
  DemuxB/3 -> P1/2, N2/2

== system beaver_agent_env_ground_static_preserved/GroundContactTireSteering/ThreePointGroundDynamics/RightMainGear/ContactGeometry/UncompressedPointRotationVelocity ==
  A : Inport
  B : Inport  Port=2
  C1 : Sum  Inputs=+-
  C2 : Sum  Inputs=+-
  C3 : Sum  Inputs=+-
  DemuxA : Demux  Outputs=3
  DemuxB : Demux  Outputs=3
  N1 : Product  Inputs=**
  N2 : Product  Inputs=**
  N3 : Product  Inputs=**
  P1 : Product  Inputs=**
  P2 : Product  Inputs=**
  P3 : Product  Inputs=**
  Result : Mux  Inputs=3
  AxB : Outport
  wires:
  Result/1 -> AxB/1
  P3/1 -> C3/1
  C3/1 -> Result/3
  C2/1 -> Result/2
  P2/1 -> C2/1
  DemuxB/1 -> P2/2, N3/2
  C1/1 -> Result/1
  N3/1 -> C3/2
  N2/1 -> C2/2
  DemuxA/3 -> N1/1, P2/1
  N1/1 -> C1/2
  P1/1 -> C1/1
  B/1 -> DemuxB/1
  A/1 -> DemuxA/1
  DemuxA/1 -> N2/1, P3/1
  DemuxB/2 -> N1/2, P3/2
  DemuxB/3 -> P1/2, N2/2
  DemuxA/2 -> P1/1, N3/1
